simulink model "shiyan4_2"  (R2021b)
settings: Solver=ode45  StartTime=0.0  StopTime=500/synFr  FixedStep=1/(3*synFr*synN/synM)  MaxStep=.4/(synFr*synN)  RelTol=1e-3  EnableMultiTasking=on
PreLoadFcn:
  | synM=.3;    % Fractional factor
  | synN=10;    % Fractional factor
  | synFr=1e7;   % Reference frequency
  | synFq=9e7;   % VCO quiescent frequency
  | synSen=1e7;   % VCO sensitivity
undefined symbols (not defined in the file): slcm
libraries: dsparch4 x1, commsynccomp2 x1
CloseFcn:
  | clear synM synN synFr synFq synSen synSigsOut
settings Model: Creator=ysong  LastModifiedBy=QYC
settings SolverCC: InitialStep=.4/(synFr*synN)  AlgebraicLoopSolver=TrustRegion
settings DataIOCC: SaveFormat=Array  SignalLoggingSaveFormat=ModelDataLogs  SaveOutput=off  SaveTime=off  ReturnWorkspaceOutputs=off  SignalLoggingName=synSigsOut
settings OptimizationCC: BlockReduction=off  BooleanDataType=off  OptimizeBlockIOStorage=off  BufferReuse=off  GlobalBufferReuse=off  ExpressionFolding=off  LocalBlockOutputs=off  InitFltsAndDblsToZero=on  OptimizeDataStoreBuffers=off  BusAssignmentInplaceUpdate=off
settings DebuggingCC: SaveWithParameterizedLinksMsg=none  UnderspecifiedInitializationDetection=Classic  MergeDetectMultiDrivingBlocksExec=none  MultiTaskDSMMsg=warning  MultiTaskCondExecSysMsg=none  SFUnexpectedBacktrackingDiag=warning  SFNoUnconditionalDefaultTransitionDiag=warning  SFExecutionAtInitializationDiag=none  SFMachineParentedDataDiag=warning  ArithmeticOperatorsInVariantConditions=warning
settings HardwareCC: ProdBitPerPointer=32  ProdBitPerSizeT=32  ProdBitPerPtrDiffT=32  ProdLargestAtomicFloat=None  ProdIntDivRoundTo=Undefined  ProdEndianess=Unspecified  ProdWordSize=32  ProdHWDeviceType=32-bit Generic  TargetUnknown=on
settings ModelReferenceCC: UpdateModelReferenceTargets=IfOutOfDate  PropagateSignalLabelsOutOfModel=off
settings SFSimCC: SimUseLocalCustomCode=off  CustomCodeUndefinedFunction=UseInterfaceOnly
settings RTWCC: RTWUseLocalCustomCode=off
settings CodeAppCC: StateflowObjectComments=on
settings GRTTargetCC: TargetFcnLib=ansi_tfl_tmw.mat  TargetLangStandard=C89/C90 (ANSI)  CombineOutputUpdateFcns=off  GRTInterface=on
settings ConfigComp: CovMetricSettings=d  CovSaveCumulativeToWorkspaceVar=on  CovSaveSingleToWorkspaceVar=on  CovExternalEMLEnable=off

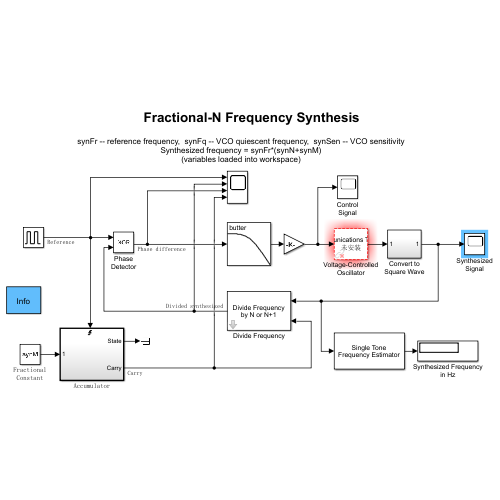
[thumbnail: Simulink's stored preview of the top-level diagram]
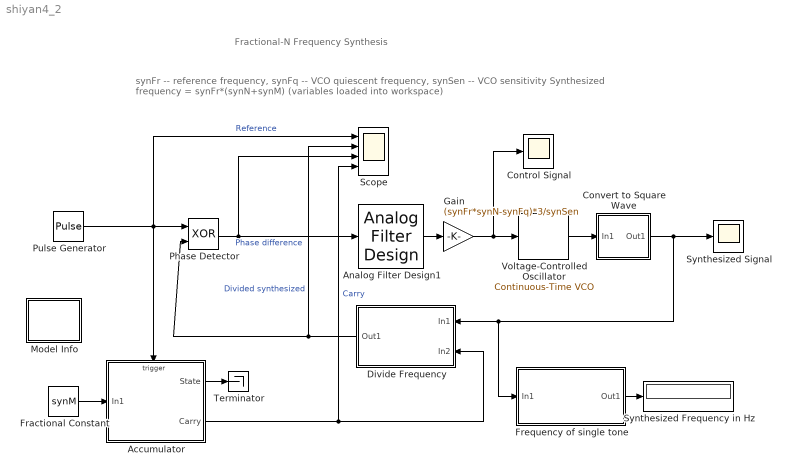
== system shiyan4_2 ==
  note: Fractional-N Frequency Synthesis
  note: synFr -- reference frequency,  synFq -- VCO quiescent frequency,  synSen -- VCO sensitivity
      | Synthesized frequency = synFr*(synN+synM)
      | (variables loaded into workspace)
  Accumulator : Subsystem  TreatAsAtomicUnit=on
  Analog Filter Design1 : dsparch4/Analog Filter Design  method=Butterworth  filttype=Lowpass  N=1  Wlo=synFr/15  Whi=80  Rp=2  Rs=40
  Control Signal : Scope
  Convert to Square Wave : Subsystem
  Divide Frequency : Subsystem  mask(Divide frequency by N or N+1){N=synN}
      mask help: Divide input frequency by N or N+1 depending on the control port.
      mask Display: disp(['Divide Frequency\nby N or N+1']);
  Fractional Constant : Constant  Value=synM
  Frequency of single tone : Subsystem
      mask Display: disp('Single Tone\nFrequency Estimator');
  Gain : Gain  Gain=(synFr*synN-synFq)*3/synSen  SaturateOnIntegerOverflow=on  OutDataTypeStr=Inherit: Same as input  ParamDataTypeStr=Inherit: Same as input
  Model Info : Subsystem  LoadFcn=slcm LoadBlock;  InitFcn=slcm('UpdateAllCMBlocksInThisModelInit')  mask(CMBlock){InitialSaveTempField=, InitialBlockCM=none, BlockCM=none, Frame=on, SaveTempField=, DisplayStringWithTags=Info, MaskDisplayString=Info, HorizontalTextAlignment=Center, LeftAlignmentValue=0.5, SourceBlockDiagram=fracsyn, TagMaxNumber=20, CMTag1=, CMTag2=, CMTag3=, CMTag4=, CMTag5=, CMTag6=, CMTag7=, CMTag8=, CMTag9=, CMTag10=, CMTag11=, CMTag12=, CMTag13=, CMTag14=, CMTag15=, CMTag16=, CMTag17=, CMTag18=, CMTag19=, CMTag20=}
      mask help: This block allows revision control information to be displayed within the model.
      settings: CopyFcn=slcm CopyBlock;  DeleteFcn=slcm Cancel;  PostSaveFcn=slcm('UpdateAllCMBlocksInThisModel')  NameChangeFcn=slcm Rename;  OpenFcn=commdemohelp;
      mask Display: text(str2num(LeftAlignmentValue), 0.5, MaskDisplayString, 'HorizontalAlignment', HorizontalTextAlignment)
  Phase Detector : Logic  Operator=XOR
  Pulse Generator : DiscretePulseGenerator  PulseType=Time based  Period=1/synFr  PulseWidth=50
  Scope : Scope  NumInputPorts=4
  Synthesized Signal : Scope
  Synthesized Frequency in Hz : Display
  Terminator : Terminator
  Voltage-Controlled Oscillator : commsynccomp2/Continuous-Time VCO  Ac=1  Fc=synFq  Kc=synSen  Ph=0
      settings: SourceProductBaseCode=CM
  wires:
  Divide Frequency/1(Out1) -> Phase Detector/2, Scope/2  "Divided synthesized"
  Gain/1 -> Control Signal/1, Voltage-Controlled Oscillator/1
  Voltage-Controlled Oscillator/1 -> Convert to Square Wave/1(In1)
  Phase Detector/1 -> Analog Filter Design1/1, Scope/3  "Phase difference"
  Convert to Square Wave/1(Out1) -> Synthesized Signal/1, Divide Frequency/1(In1), Frequency of single tone/1(In1)
  Frequency of single tone/1(Out1) -> Synthesized Frequency in Hz/1
  Accumulator/1(State) -> Terminator/1
  Accumulator/2(Carry) -> Divide Frequency/2(In2), Scope/4  "Carry"
  Pulse Generator/1 -> Phase Detector/1, Scope/1, Accumulator/Trigger  "Reference"
  Fractional Constant/1 -> Accumulator/1(In1)
  Analog Filter Design1/1 -> Gain/1

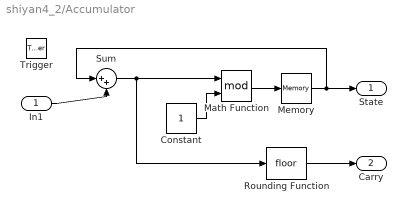
== system shiyan4_2/Accumulator ==
  In1 : Inport
  Trigger : TriggerPort  VariantControl=(inherit)  ZeroCross=off
  Constant : Constant
  Math Function : Math  Operator=mod  SignedPower=on  SaturateOnIntegerOverflow=on
  Memory : Memory  InheritSampleTime=on
  Rounding Function : Rounding
  Sum : Sum  Inputs=|++  InputSameDT=on  SaturateOnIntegerOverflow=on  OutDataTypeStr=Inherit: Same as first input
  State : Outport  VectorParamsAs1DForOutWhenUnconnected=off
  Carry : Outport  Port=2  VectorParamsAs1DForOutWhenUnconnected=off
  wires:
  Constant/1 -> Math Function/2
  In1/1 -> Sum/2
  Memory/1 -> Sum/1, State/1
  Sum/1 -> Math Function/1, Rounding Function/1
  Math Function/1 -> Memory/1
  Rounding Function/1 -> Carry/1

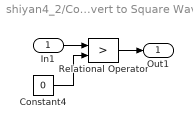
== system shiyan4_2/Convert to Square Wave ==
  In1 : Inport
  Constant4 : Constant  Value=0
  Relational Operator : RelationalOperator  Operator=>  RndMeth=Nearest  InputSameDT=on
  Out1 : Outport  VectorParamsAs1DForOutWhenUnconnected=off
  wires:
  Relational Operator/1 -> Out1/1
  In1/1 -> Relational Operator/1
  Constant4/1 -> Relational Operator/2

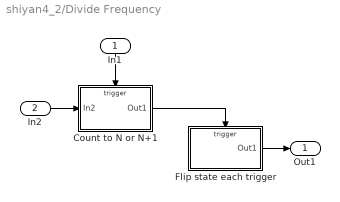
== system shiyan4_2/Divide Frequency ==
  In1 : Inport
  In2 : Inport  Port=2
  Count to N or N+1 : Subsystem  TreatAsAtomicUnit=on
  Flip state each trigger : Subsystem  TreatAsAtomicUnit=on
  Out1 : Outport  VectorParamsAs1DForOutWhenUnconnected=off
  wires:
  Count to N or N+1/1(Out1) -> Flip state each trigger/Trigger
  Flip state each trigger/1(Out1) -> Out1/1
  In1/1 -> Count to N or N+1/Trigger
  In2/1 -> Count to N or N+1/1(In2)

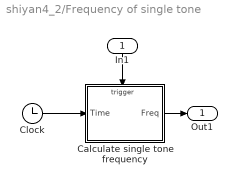
== system shiyan4_2/Frequency of single tone ==
  In1 : Inport
  Calculate single tone frequency : Subsystem  TreatAsAtomicUnit=on
  Clock : Clock
  Out1 : Outport  VectorParamsAs1DForOutWhenUnconnected=off
  wires:
  In1/1 -> Calculate single tone frequency/Trigger
  Clock/1 -> Calculate single tone frequency/1(Time)
  Calculate single tone frequency/1(Freq) -> Out1/1

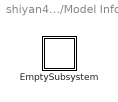
== system shiyan4_2/Model Info ==
  EmptySubsystem : Subsystem

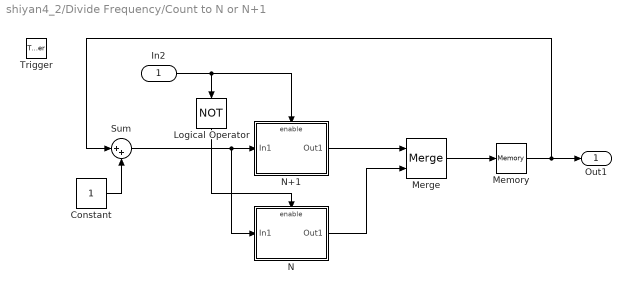
== system shiyan4_2/Divide Frequency/Count to N or N+1 ==
  In2 : Inport
  Trigger : TriggerPort  TriggerType=either  VariantControl=(inherit)  ZeroCross=off
  Constant : Constant
  Logical Operator : Logic  Operator=NOT
  Memory : Memory  InitialCondition=1  InheritSampleTime=on
  Merge : Merge
  N : Subsystem  TreatAsAtomicUnit=on
  N+1 : Subsystem  TreatAsAtomicUnit=on
  Sum : Sum  Inputs=|++  InputSameDT=on  SaturateOnIntegerOverflow=on  OutDataTypeStr=Inherit: Same as first input
  Out1 : Outport  VectorParamsAs1DForOutWhenUnconnected=off
  wires:
  Logical Operator/1 -> N/Enable
  In2/1 -> Logical Operator/1, N+1/Enable
  N+1/1(Out1) -> Merge/1
  N/1(Out1) -> Merge/2
  Merge/1 -> Memory/1
  Constant/1 -> Sum/2
  Sum/1 -> N+1/1(In1), N/1(In1)
  Memory/1 -> Sum/1, Out1/1

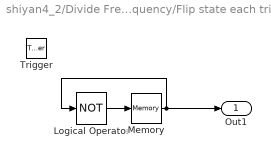
== system shiyan4_2/Divide Frequency/Flip state each trigger ==
  Trigger : TriggerPort  TriggerType=falling  VariantControl=(inherit)  ZeroCross=off
  Logical Operator : Logic  Operator=NOT
  Memory : Memory  InitialCondition=1  InheritSampleTime=on
  Out1 : Outport  InitialOutput=0  VectorParamsAs1DForOutWhenUnconnected=off
  wires:
  Logical Operator/1 -> Memory/1
  Memory/1 -> Out1/1, Logical Operator/1

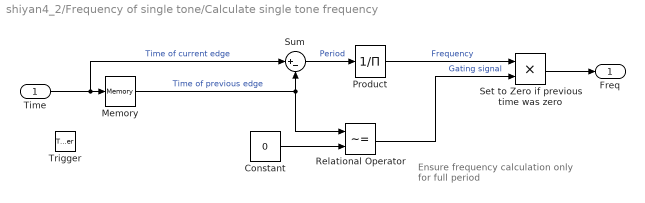
== system shiyan4_2/Frequency of single tone/Calculate single tone frequency ==
  note: Ensure frequency calculation
      | only for full period
  Time : Inport
  Trigger : TriggerPort  VariantControl=(inherit)  ZeroCross=off
  Constant : Constant  Value=0
  Memory : Memory  InheritSampleTime=on
  Product : Product  Inputs=/  InputSameDT=on  SaturateOnIntegerOverflow=on  OutDataTypeStr=Inherit: Same as first input
  Relational Operator : RelationalOperator  Operator=~=  RndMeth=Nearest  InputSameDT=on
  Set to Zero if previous time was zero : Product  InputSameDT=on  SaturateOnIntegerOverflow=on  OutDataTypeStr=Inherit: Same as first input
  Sum : Sum  Inputs=|+-  InputSameDT=on  SaturateOnIntegerOverflow=on  OutDataTypeStr=Inherit: Same as first input
  Freq : Outport  InitialOutput=0  VectorParamsAs1DForOutWhenUnconnected=off
  wires:
  Time/1 -> Sum/1, Memory/1  "Time of current edge"
  Sum/1 -> Product/1  "Period"
  Product/1 -> Set to Zero if previous time was zero/1  "Frequency"
  Memory/1 -> Sum/2, Relational Operator/1  "Time of previous edge"
  Set to Zero if previous time was zero/1 -> Freq/1
  Constant/1 -> Relational Operator/2
  Relational Operator/1 -> Set to Zero if previous time was zero/2  "Gating signal"

== system shiyan4_2/Model Info/EmptySubsystem ==

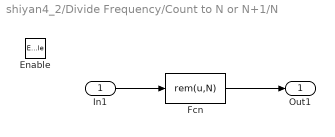
== system shiyan4_2/Divide Frequency/Count to N or N+1/N ==
  In1 : Inport
  Enable : EnablePort  ZeroCross=off
  Fcn : Fcn  Expr=rem(u,N)
  Out1 : Outport  VectorParamsAs1DForOutWhenUnconnected=off
  wires:
  Fcn/1 -> Out1/1
  In1/1 -> Fcn/1

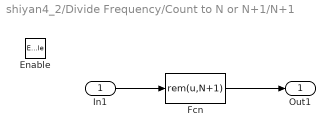
== system shiyan4_2/Divide Frequency/Count to N or N+1/N+1 ==
  In1 : Inport
  Enable : EnablePort  ZeroCross=off
  Fcn : Fcn  Expr=rem(u,N+1)
  Out1 : Outport  VectorParamsAs1DForOutWhenUnconnected=off
  wires:
  In1/1 -> Fcn/1
  Fcn/1 -> Out1/1
